simulink model "TV_Sim_Track_Copia"  (R2025b)
settings: Solver=VariableStepAuto  StartTime=0.0  StopTime=20  RelTol=1e-3
values from neighbouring files (symbols this model uses):
  Ki_array = zeros(size(Vx_array))    [PID_analysis.m]    (also in PID_tuning.m)
  psi_ref = theta + pi/2    [init_skidpad.m]
  s_ref = linspace(0, circonferenza, 200)    [init_skidpad.m]
  Vx_array = 1:1:30    [PID_analysis.m]    (also in PID_tuning.m)
  x_ref = R * cos(theta)    [init_skidpad.m]
  y_ref = R * sin(theta)    [init_skidpad.m]
undefined symbols (not defined in the file or in its folder): vp
libraries: slpidlib x3
(part 2 of 2)

== matlab function TV_Sim_Track_Copia/MATLAB Function6 ==
  data: T_RL_req input; T_RL_out output; T_RR_req input; T_RR_out output; omega_RL input; omega_RR input; u input; vp parameter
function [T_RL_out, T_RR_out] = ASC_Controller(T_RL_req, T_RR_req, omega_RL, omega_RR, u, vp)
    % TARGET
    % Poiché la tua formula dà slip negativo in accelerazione,
    % usiamo il valore assoluto per semplificare il confronto.
    target_slip_abs = -0.11; 
    K_p = 500;
    
    % Raggio ruota
    R = vp.Rr;

    % --- RUOTA POSTERIORE SINISTRA ---
    V_wheel_RL = omega_RL * R;
    
    % Protezione divisione per zero (Se la ruota è quasi ferma, slip è 0)
    if abs(V_wheel_RL) < 0.1
        slip_RL = 0;
    else
        % TUA FORMULA: (u - Vr) / Vr
        slip_RL = (u - V_wheel_RL) / V_wheel_RL;
    end
    
    % Logica di controllo con Valore Assoluto
    % Nota: In accelerazione slip_RL sarà negativo (es. -0.2).
    % abs(-0.2) = 0.2, che è > 0.15 -> INTERVIENE IL CONTROLLO
    if slip_RL < target_slip_abs
        
        % Calcoliamo l'errore in valore assoluto
        error_slip = target_slip_abs - slip_RL;
        
        % Tagliamo la coppia
        T_cut = error_slip * K_p;
        T_RL_out = T_RL_req - T_cut;
        
    else
        T_RL_out = T_RL_req;
    end

    % Protezione
    if T_RL_out < -vp.Tregenmax; T_RL_out = -vp.Tregenmax; end
    
    % --- RUOTA POSTERIORE DESTRA (Idem) ---
    V_wheel_RR = omega_RR * R;
    
    if abs(V_wheel_RR) < 0.1
        slip_RR = 0;
    else
        slip_RR = (u - V_wheel_RR) / V_wheel_RR;
    end
    
    if slip_RR < target_slip_abs
        error_slip = target_slip_abs - slip_RR;
        T_cut = error_slip * K_p;
        T_RR_out = T_RR_req - T_cut;
        
    else
        T_RR_out = T_RR_req;
    end

    if T_RR_out < -vp.Tregenmax; T_RR_out = -vp.Tregenmax; end
end

== matlab function TV_Sim_Track_Copia/MATLAB Function7 ==
  data: v_target output
function v_target = fcn()
    g = 9.81; % Accelerazione di gravità
    R = 9.125;
    curvatura = 1/R;
    mu = 0.9; 
    % 1. Calcolo della velocità limite fisica (Velocità Critica)
    % Usiamo un piccolo valore (eps) per evitare la divisione per zero in rettilineo
    if abs(curvatura) > 0.0001
        v_limite = sqrt((mu * g) / abs(curvatura));
    else
        v_limite = 250 / 3.6; % In rettilineo, limite massimo (es. 250 km/h)
    end
    
    % 2. Fattore di sicurezza (Pilota)
    % Un pilota umano non sta al 100.0% del limite o l'auto scivola.
    % Usiamo il 95% del limite fisico.
    v_target = v_limite * 0.95;
    
    % 3. Gestione della frenata (Anticipazione)
    % Se la velocità target è molto più bassa di quella attuale, 
    % il segnale passerà al PID che comanderà coppia negativa (freno).
end

== matlab function TV_Sim_Track_Copia/MATLAB Function8 ==
  data: v_target output
function v_target = fcn()
    g = 9.81; % Accelerazione di gravità
    R = 9.125;
    curvatura = 1/R;
    mu = 0.9; 
    % 1. Calcolo della velocità limite fisica (Velocità Critica)
    % Usiamo un piccolo valore (eps) per evitare la divisione per zero in rettilineo
    if abs(curvatura) > 0.0001
        v_limite = sqrt((mu * g) / abs(curvatura));
    else
        v_limite = 250 / 3.6; % In rettilineo, limite massimo (es. 250 km/h)
    end
    
    % 2. Fattore di sicurezza (Pilota)
    % Un pilota umano non sta al 100.0% del limite o l'auto scivola.
    % Usiamo il 95% del limite fisico.
    v_target = v_limite * 0.95;
    
    % 3. Gestione della frenata (Anticipazione)
    % Se la velocità target è molto più bassa di quella attuale, 
    % il segnale passerà al PID che comanderà coppia negativa (freno).
end

== matlab function TV_Sim_Track_Copia/Subsystem2/MATLAB Function10 ==
  data: e_ct input; delta_out output; theta_e input; v input; psi_ref_vector input; W input
function delta_out  = fcn(e_ct, theta_e, v, psi_ref_vector, W)
    % --- PARAMETRI DI CONFIGURAZIONE ---
    N = length(psi_ref_vector); % Numero di punti futuri (es. 10)
    dt = 0.1;                   % Passo temporale della previsione [s]
    L = 2.5;                    % Interasse del veicolo [m]
    
    % Margine di sicurezza: l'auto cercherà di stare entro questo limite
    % Se W=10m, Lat_Limit sarà 4.7m (lasciando 30cm dal bordo)
    Lat_Limit = (W/2) - 0.3; 

    % --- 1. PREVISIONE DEL FUTURO (ORIZZONTE N) ---
    % Inizializziamo le variabili per la simulazione interna
    future_e_ct = zeros(1, N);
    temp_e = e_ct;
    temp_theta = theta_e;
    
for k = 1:N
    % Calcola la differenza angolare
    diff_angle = temp_theta - psi_ref_vector(k);
    
    % CORREZIONE WRAP-AROUND: mantiene l'angolo tra -pi e pi
    diff_angle = atan2(sin(diff_angle), cos(diff_angle));
    
    % Usa l'angolo corretto per la previsione
    temp_e = temp_e + v * sin(diff_angle) * dt;
    future_e_ct(k) = temp_e;
end

    % --- 2. LOGICA DI CONTROLLO STERZO (FEEDBACK) ---
    % Usiamo una base simile allo Stanley per l'inseguimento normale
    k_stanley = 0.5;
    k_soft = 1.0;
    delta_feedback = theta_e - atan2(k_stanley * e_ct, v + k_soft);

    % --- 3. LOGICA DI VINCOLO (THE "HARD" CONSTRAINT) ---
    % Troviamo l'errore massimo previsto nell'orizzonte
    max_predicted_error = max(abs(future_e_ct));
    
    if max_predicted_error > Lat_Limit
        % --- SE L'AUTO PREVEDE DI USCIRE ---
        
        % A. Calcoliamo quanto stiamo violando il limite
        violazione = max_predicted_error - Lat_Limit;
     
        % C. STERZO DI EMERGENZA: Aumentiamo il guadagno per chiudere la curva
        delta_out = delta_feedback * (1 + 2 * violazione);
    else
        % --- TRAIETTORIA SICURA ---
        delta_out = delta_feedback;
    end

    % --- 4. SATURAZIONI FISICHE ---
    % Limite sterzo (es. 35 gradi)
    delta_out = max(min(delta_out, 0.6), -0.6);
end
